simulink model "Network_Subsystem"  (R2025a)
settings: Solver=ode45  StartTime=0.0  StopTime=86400  MaxStep=1e-4  MinStep=1e-8  RelTol=1e-5  AbsTol=1e-8
settings Model: Creator=denis  LastModifiedBy=denis

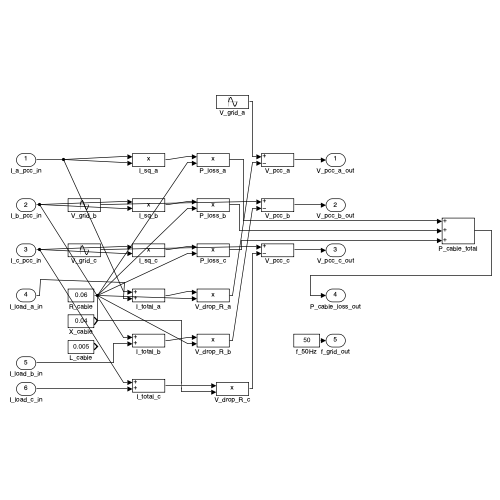
[thumbnail: Simulink's stored preview of the top-level diagram]
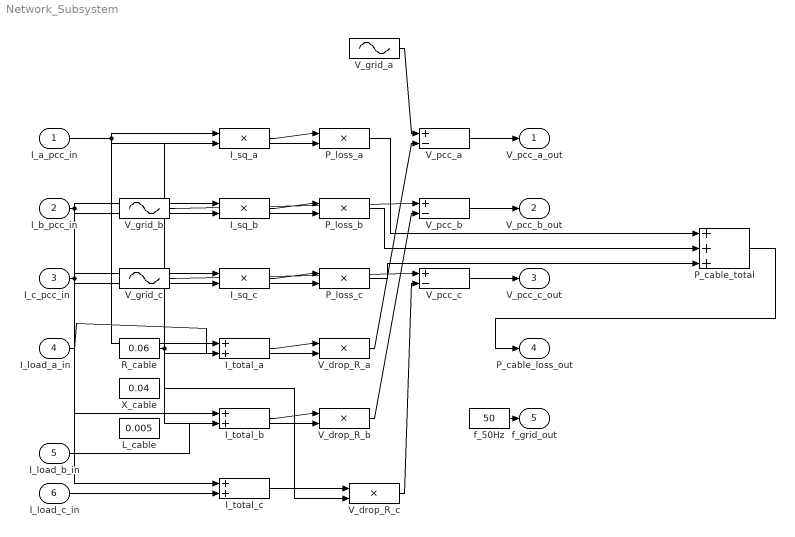
== system Network_Subsystem ==
  I_a_pcc_in : Inport
  I_b_pcc_in : Inport  Port=2
  I_c_pcc_in : Inport  Port=3
  I_load_a_in : Inport  Port=4
  I_load_b_in : Inport  Port=5
  I_load_c_in : Inport  Port=6
  I_sq_a : Product
  I_sq_b : Product
  I_sq_c : Product
  I_total_a : Sum
  I_total_b : Sum
  I_total_c : Sum
  L_cable : Constant  Value=0.005
  P_cable_total : Sum  Inputs=+++
  P_loss_a : Product
  P_loss_b : Product
  P_loss_c : Product
  R_cable : Constant  Value=0.06
  V_drop_R_a : Product
  V_drop_R_b : Product
  V_drop_R_c : Product
  V_grid_a : Sin  Amplitude=5773.5  Frequency=50  SampleTime=0
  V_grid_b : Sin  Amplitude=5773.5  Frequency=50  Phase=-2.0944  SampleTime=0
  V_grid_c : Sin  Amplitude=5773.5  Frequency=50  Phase=2.0944  SampleTime=0
  V_pcc_a : Sum  Inputs=+-
  V_pcc_b : Sum  Inputs=+-
  V_pcc_c : Sum  Inputs=+-
  X_cable : Constant  Value=0.04
  f_50Hz : Constant  Value=50
  V_pcc_a_out : Outport
  V_pcc_b_out : Outport  Port=2
  V_pcc_c_out : Outport  Port=3
  P_cable_loss_out : Outport  Port=4
  f_grid_out : Outport  Port=5
  wires:
  I_a_pcc_in/1 -> I_sq_a/1, I_sq_a/2, I_total_a/1
  I_sq_a/1 -> P_loss_a/1
  R_cable/1 -> P_loss_a/2, P_loss_b/2, P_loss_c/2, V_drop_R_a/2, V_drop_R_b/2, V_drop_R_c/2
  I_b_pcc_in/1 -> I_sq_b/1, I_sq_b/2, I_total_b/1
  I_sq_b/1 -> P_loss_b/1
  I_c_pcc_in/1 -> I_sq_c/1, I_sq_c/2, I_total_c/1
  I_sq_c/1 -> P_loss_c/1
  P_loss_a/1 -> P_cable_total/1
  P_loss_b/1 -> P_cable_total/2
  P_loss_c/1 -> P_cable_total/3
  I_load_a_in/1 -> I_total_a/2
  I_load_b_in/1 -> I_total_b/2
  I_load_c_in/1 -> I_total_c/2
  I_total_a/1 -> V_drop_R_a/1
  I_total_b/1 -> V_drop_R_b/1
  I_total_c/1 -> V_drop_R_c/1
  V_grid_a/1 -> V_pcc_a/1
  V_drop_R_a/1 -> V_pcc_a/2
  V_grid_b/1 -> V_pcc_b/1
  V_drop_R_b/1 -> V_pcc_b/2
  V_grid_c/1 -> V_pcc_c/1
  V_drop_R_c/1 -> V_pcc_c/2
  V_pcc_a/1 -> V_pcc_a_out/1
  V_pcc_b/1 -> V_pcc_b_out/1
  V_pcc_c/1 -> V_pcc_c_out/1
  P_cable_total/1 -> P_cable_loss_out/1
  f_50Hz/1 -> f_grid_out/1
